simulink model "Three_Stages"  (R2023a)
settings: Solver=FixedStepDiscrete  StartTime=0.0  StopTime=5000  FixedStep=1  RelTol=1e-3
values from neighbouring files (symbols this model uses):
  fw = zeros(16384, 1, 'uint32')    [test.m]
libraries: hdlsllib x27, simulink x27, etargetslib x1
(part 1 of 5)
settings Model: PauseTimes=9  Creator=11983  LastModifiedBy=11983

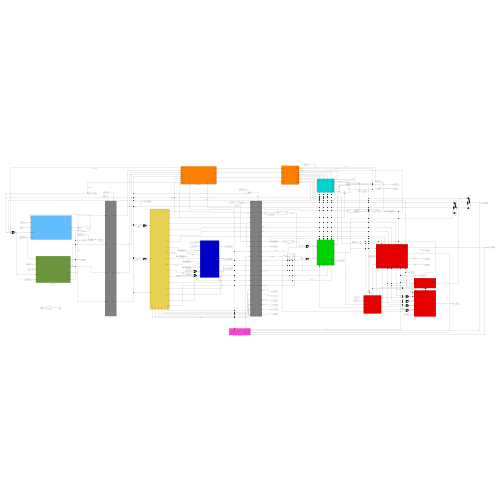
[thumbnail: Simulink's stored preview of the top-level diagram]
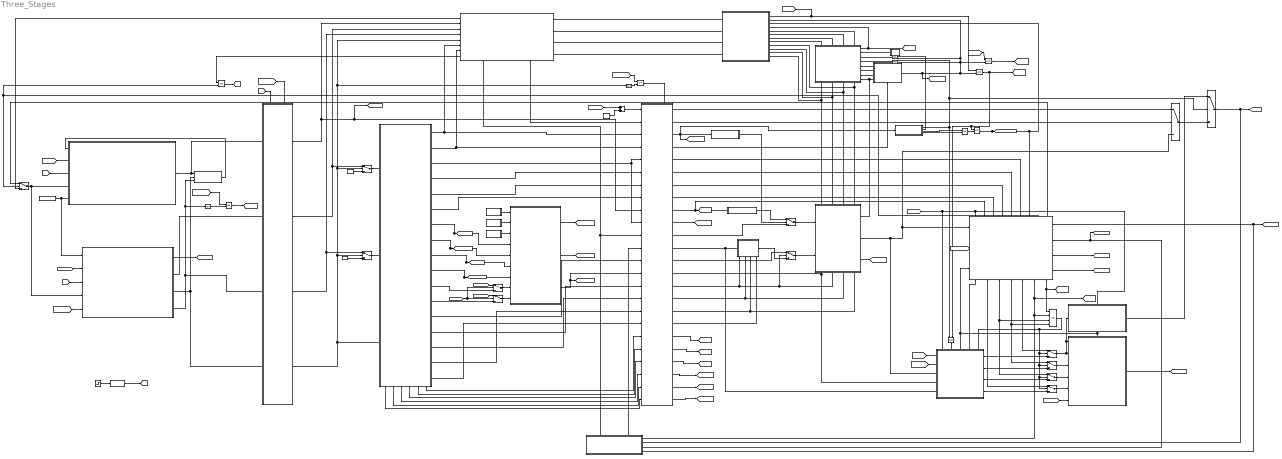
== system Three_Stages ==
  ALU : Subsystem
      settings: PortSchema="{\"entries\":[{\"content\":{\"sides\":[{\"content\":{\"connectorIds\":[\"In1\",\"In2\"]},\"type\":\"ConnectorPlacement.EquallySpacedRectSide\",\"uuid\":\"ccb5df41-1247-48d9-959c-75926096b8fa\"},{\"content\":{\"connectorIds\":[\"In7\",\"Out1\",\"Out2\"],\"side\":\"RIGHT\"},\"type\":\"ConnectorPlacement.EquallySpacedRectSide\",\"uuid\":\"80f2a142-6d0c-48b1-ae68-4f85aa7180f9\"},{\"content\":{\"connectorIds\":[\"Out3\",\"Out4\",\"Out5\",\"Out6\"],\"side\":\"TOP\"},\"type\":\"ConnectorPlacement.EquallySpacedRectSide\",\"uuid\":\"ddd8a3a0-1a29-4746-aba9-d3a66e616423\"},{\"content\":{\"connectorIds\":[\"In3\",\"In4\",\"In5\",\"In6\"],\"side\":\"BOTTOM\"},\"type\":\"ConnectorPlacement.EquallySpacedRectSide\",\"uuid\":\"5581b6e8-dec6-4a13-b9b3-e754e41154dd\"}]},\"type\":\"ConnectorPlacement.EquallySpacedConnector\",\"uuid\":\"f4739204-0172-45d8-8900-7f7503b7c069\"}],\"packageUris\":[\"http://schema.mathworks.com/mf0/Connector/R2020b\"],\"version\":\"1.0\"}"
  APSR : Subsystem
      settings: PortSchema="{\"entries\":[{\"content\":{\"sides\":[{\"content\":{},\"type\":\"ConnectorPlacement.EquallySpacedRectSide\",\"uuid\":\"b04420ff-f19b-4c94-a003-74643939b36f\"},{\"content\":{\"connectorIds\":[\"In5\",\"In6\",\"In7\",\"In8\",\"Out1\",\"Out2\",\"Out3\",\"Out4\"],\"side\":\"RIGHT\"},\"type\":\"ConnectorPlacement.EquallySpacedRectSide\",\"uuid\":\"262487a7-9547-4f2e-9b3b-f72102858df0\"},{\"content\":{\"connectorIds\":[\"Out5\",\"Out6\",\"Out7\",\"Out8\"],\"side\":\"TOP\"},\"type\":\"ConnectorPlacement.EquallySpacedRectSide\",\"uuid\":\"08655cd2-da14-4b4c-a3be-8f888e927bf2\"},{\"content\":{\"connectorIds\":[\"In1\",\"In2\",\"In3\",\"In4\"],\"side\":\"BOTTOM\"},\"type\":\"ConnectorPlacement.EquallySpacedRectSide\",\"uuid\":\"d1ff2338-8405-4e4f-9e8f-6e9f9acda6a4\"}]},\"type\":\"ConnectorPlacement.EquallySpacedConnector\",\"uuid\":\"02373ca2-1c43-4ba4-bf90-ab64c05b49a0\"}],\"packageUris\":[\"http://schema.mathworks.com/mf0/Connector/R2020b\"],\"version\":\"1.0\"}"
  Add : Sum
  Branch_Unit : Subsystem
      settings: PortSchema="{\"entries\":[{\"content\":{\"sides\":[{\"content\":{\"connectorIds\":[\"Out2\",\"In1\",\"In2\",\"In3\",\"In4\",\"In5\",\"In6\",\"Out3\"]},\"type\":\"ConnectorPlacement.EquallySpacedRectSide\",\"uuid\":\"fa39de6f-023a-4353-bbb3-beec0acef9a4\"},{\"content\":{\"connectorIds\":[\"In8\",\"In9\",\"In10\",\"In11\"],\"side\":\"RIGHT\"},\"type\":\"ConnectorPlacement.EquallySpacedRectSide\",\"uuid\":\"2cd56a38-3fbf-451b-a1e9-9297fd516597\"},{\"content\":{\"side\":\"TOP\"},\"type\":\"ConnectorPlacement.EquallySpacedRectSide\",\"uuid\":\"e24db981-f1ca-4813-8aa8-2d70266521c8\"},{\"content\":{\"connectorIds\":[\"In7\",\"Out1\"],\"side\":\"BOTTOM\"},\"type\":\"ConnectorPlacement.EquallySpacedRectSide\",\"uuid\":\"8566e1d9-99e4-42a3-b963-6f1483e5acef\"}]},\"type\":\"ConnectorPlacement.EquallySpacedConnector\",\"uuid\":\"2efaa27e-3a9b-48f9-ab74-8d4ce9e9e835\"}],\"packageUris\":[\"http://schema.mathworks.com/mf0/Connector/R2020b\"],\"version\":\"1.0\"}"
  COND_OK : Subsystem
      settings: PortSchema="{\"entries\":[{\"content\":{\"sides\":[{\"content\":{\"connectorIds\":[\"In1\",\"In2\",\"In3\",\"In4\"]},\"type\":\"ConnectorPlacement.EquallySpacedRectSide\",\"uuid\":\"b7de4efa-7ffd-4508-af86-f3994ca8b638\"},{\"content\":{\"connectorIds\":[\"Out1\"],\"side\":\"RIGHT\"},\"type\":\"ConnectorPlacement.EquallySpacedRectSide\",\"uuid\":\"01c63998-7571-4d66-95c8-a8f2c37a5aa2\"},{\"content\":{\"side\":\"TOP\"},\"type\":\"ConnectorPlacement.EquallySpacedRectSide\",\"uuid\":\"ed1382b1-aa61-428b-a7ef-96829cef3c86\"},{\"content\":{\"connectorIds\":[\"In5\"],\"side\":\"BOTTOM\"},\"type\":\"ConnectorPlacement.EquallySpacedRectSide\",\"uuid\":\"571a99ab-d0c2-4e4e-a524-83c5ee223b5b\"}]},\"type\":\"ConnectorPlacement.EquallySpacedConnector\",\"uuid\":\"3f5959c9-782a-410f-ad4b-6735c3db51ba\"}],\"packageUris\":[\"http://schema.mathworks.com/mf0/Connector/R2020b\"],\"version\":\"1.0\"}"
  Constant : Constant  Value=0  OutDataTypeStr=uint32
  Constant1 : Constant  Value=0
  Constant3 : Constant  Value=0x08000130  VectorParams1D=off
  Constant7 : Constant  Value=4  OutDataTypeStr=uint32
  Data Type Conversion : DataTypeConversion  OutDataTypeStr=boolean  SaturateOnIntegerOverflow=off  RndMeth=Floor
  Forward_Unit : Subsystem
      settings: PortSchema="{\"entries\":[{\"content\":{\"sides\":[{\"content\":{},\"type\":\"ConnectorPlacement.EquallySpacedRectSide\",\"uuid\":\"b518ab8e-5181-4ba3-962c-c49c8d938615\"},{\"content\":{\"connectorIds\":[\"In1\",\"In2\",\"In3\",\"In4\"],\"side\":\"RIGHT\"},\"type\":\"ConnectorPlacement.EquallySpacedRectSide\",\"uuid\":\"5317ce62-8cb4-48f5-b950-79d5c38b61e0\"},{\"content\":{\"connectorIds\":[\"Out1\",\"Out2\"],\"side\":\"TOP\"},\"type\":\"ConnectorPlacement.EquallySpacedRectSide\",\"uuid\":\"43e255fe-bf02-429e-afe6-23a00690485d\"}]},\"type\":\"ConnectorPlacement.EquallySpacedConnector\",\"uuid\":\"73139baf-ff19-4893-8dbb-73622a3eec4b\"}],\"packageUris\":[\"http://schema.mathworks.com/mf0/Connector/R2020b\"],\"version\":\"1.0\"}"
  LDRB_LDRH : Subsystem
      settings: PortSchema="{\"entries\":[{\"content\":{\"sides\":[{\"content\":{\"connectorIds\":[\"In1\"]},\"type\":\"ConnectorPlacement.EquallySpacedRectSide\",\"uuid\":\"1aacb863-4f6f-4fe7-b69a-d5773680006a\"},{\"content\":{\"connectorIds\":[\"Out1\"],\"side\":\"RIGHT\"},\"type\":\"ConnectorPlacement.EquallySpacedRectSide\",\"uuid\":\"1b0cc9e8-d7ed-4611-b678-703fc229f153\"},{\"content\":{\"connectorIds\":[\"In2\"],\"side\":\"TOP\"},\"type\":\"ConnectorPlacement.EquallySpacedRectSide\",\"uuid\":\"6cf80b36-4bc3-4f6e-89b2-b390fea3a693\"},{\"content\":{\"connectorIds\":[\"In3\"],\"side\":\"BOTTOM\"},\"type\":\"ConnectorPlacement.EquallySpacedRectSide\",\"uuid\":\"f50755aa-ce52-486e-b974-6c83f6b16ce4\"}]},\"type\":\"ConnectorPlacement.EquallySpacedConnector\",\"uuid\":\"37988c8b-84fd-4da1-be93-43b2d0148809\"}],\"packageUris\":[\"http://schema.mathworks.com/mf0/Connector/R2020b\"],\"version\":\"1.0\"}"
  LDR_Target : Subsystem
  Logical Operator{1..4,12,14} (6 alike) : Logic  AllPortsSameDT=off  OutDataTypeStr=boolean
  Logical Operator10 : Logic  Operator=OR  Inputs=4  AllPortsSameDT=off  OutDataTypeStr=boolean
  Logical Operator15 : Logic  Operator=NOT  AllPortsSameDT=off  OutDataTypeStr=boolean
  Logical Operator{5..6,21..22} (4 alike) : Logic  Operator=OR  AllPortsSameDT=off  OutDataTypeStr=boolean
  Logical Operator23 : Logic  Operator=NOT  AllPortsSameDT=off  OutDataTypeStr=boolean
  MR : Subsystem
      settings: PortSchema="{\"entries\":[{\"content\":{\"sides\":[{\"content\":{\"connectorIds\":[\"In1\",\"In2\",\"In3\"]},\"type\":\"ConnectorPlacement.EquallySpacedRectSide\",\"uuid\":\"ae034d06-3b44-4ece-97be-40f77d25c887\"},{\"content\":{\"connectorIds\":[\"Out1\",\"Out2\",\"Out3\",\"Out4\"],\"side\":\"RIGHT\"},\"type\":\"ConnectorPlacement.EquallySpacedRectSide\",\"uuid\":\"97e4f072-c582-4d8b-a0d0-105be19de914\"},{\"content\":{\"connectorIds\":[\"In4\",\"In5\",\"In6\",\"In7\",\"In8\",\"In9\",\"In10\",\"Out12\",\"Out13\"],\"side\":\"TOP\"},\"type\":\"ConnectorPlacement.EquallySpacedRectSide\",\"uuid\":\"0c52d681-aa90-4260-97f0-099fed25df92\"},{\"content\":{\"connectorIds\":[\"Out5\",\"Out6\",\"Out7\",\"Out8\",\"Out9\",\"Out10\",\"Out11\"],\"side\":\"BOTTOM\"},\"type\":\"ConnectorPlacement.EquallySpacedRectSide\",\"uuid\":\"f0439111-5f7c-4712-89ea-153c665c0054\"}]},\"type\":\"ConnectorPlacement.EquallySpacedConnector\",\"uuid\":\"3d8c92c8-6a6f-4c3f-a3c8-33ac8d15b626\"}],\"packageUris\":[\"http://schema.mathworks.com/mf0/Connector/R2020b\"],\"version\":\"1.0\"}"
  PC : Subsystem
  Prefetch_Unit : Subsystem
  Register File : Subsystem
  STRB_STRH : Subsystem
      settings: PortSchema="{\"entries\":[{\"content\":{\"sides\":[{\"content\":{\"connectorIds\":[\"In1\",\"In2\",\"In3\",\"In4\",\"In5\"]},\"type\":\"ConnectorPlacement.EquallySpacedRectSide\",\"uuid\":\"52cc573e-20cd-47d9-80c8-fb5377adebe3\"},{\"content\":{\"connectorIds\":[\"Out1\",\"Out2\",\"Out3\",\"Out4\"],\"side\":\"RIGHT\"},\"type\":\"ConnectorPlacement.EquallySpacedRectSide\",\"uuid\":\"a4a5e072-7857-4af3-85db-797d3693bf36\"},{\"content\":{\"connectorIds\":[\"In6\",\"In7\",\"In8\",\"In9\",\"In10\"],\"side\":\"TOP\"},\"type\":\"ConnectorPlacement.EquallySpacedRectSide\",\"uuid\":\"ea3ffc43-3311-4906-a9ee-9debdf9ad28c\"},{\"content\":{\"side\":\"BOTTOM\"},\"type\":\"ConnectorPlacement.EquallySpacedRectSide\",\"uuid\":\"e3f27f00-6d88-4589-b3c9-a064ef027647\"}]},\"type\":\"ConnectorPlacement.EquallySpacedConnector\",\"uuid\":\"664d1095-24c2-4b6b-a161-99b2f71d747b\"}],\"packageUris\":[\"http://schema.mathworks.com/mf0/Connector/R2020b\"],\"version\":\"1.0\"}"
  Step : Step  Time=2.2  SampleTime=1
  Subsystem1 : Subsystem
      settings: PortSchema="{\"entries\":[{\"content\":{\"sides\":[{\"content\":{\"connectorIds\":[\"In1\",\"In2\",\"In3\",\"In4\"]},\"type\":\"ConnectorPlacement.EquallySpacedRectSide\",\"uuid\":\"b636389a-7517-44e7-b701-adf22a5dae08\"},{\"content\":{\"connectorIds\":[\"Out1\",\"Out2\",\"Out3\",\"Out4\"],\"side\":\"RIGHT\"},\"type\":\"ConnectorPlacement.EquallySpacedRectSide\",\"uuid\":\"a093e9de-de32-4ec9-9bcc-d63488a9f5df\"},{\"content\":{\"connectorIds\":[\"In5\",\"In6\"],\"side\":\"TOP\"},\"type\":\"ConnectorPlacement.EquallySpacedRectSide\",\"uuid\":\"0686ded3-feaa-49de-a1b1-14e15ce2ab70\"}]},\"type\":\"ConnectorPlacement.EquallySpacedConnector\",\"uuid\":\"33f9a1b7-843e-4ab1-9626-193f0cb3215d\"}],\"packageUris\":[\"http://schema.mathworks.com/mf0/Connector/R2020b\"],\"version\":\"1.0\"}"
  Subsystem13 : Subsystem
      settings: PortSchema="{\"entries\":[{\"content\":{\"sides\":[{\"content\":{\"connectorIds\":[\"In1\"]},\"type\":\"ConnectorPlacement.EquallySpacedRectSide\",\"uuid\":\"4653521f-c5b0-44ee-87bd-1e9a678c2349\"},{\"content\":{\"connectorIds\":[\"Out1\"],\"side\":\"RIGHT\"},\"type\":\"ConnectorPlacement.EquallySpacedRectSide\",\"uuid\":\"2d3a92f1-c2bf-4739-8a2e-22a17e3c5465\"},{\"content\":{\"side\":\"TOP\"},\"type\":\"ConnectorPlacement.EquallySpacedRectSide\",\"uuid\":\"dec91679-c767-4ffa-aded-7a717f01530d\"},{\"content\":{\"connectorIds\":[\"In2\",\"In3\",\"In4\",\"In5\"],\"side\":\"BOTTOM\"},\"type\":\"ConnectorPlacement.EquallySpacedRectSide\",\"uuid\":\"b2049017-66dd-4d9f-8220-bbbb14711246\"}]},\"type\":\"ConnectorPlacement.EquallySpacedConnector\",\"uuid\":\"86f521a6-6afa-4d7d-9bc3-b40505ae83a4\"}],\"packageUris\":[\"http://schema.mathworks.com/mf0/Connector/R2020b\"],\"version\":\"1.0\"}"
  Subsystem2 : Subsystem
      settings: PortSchema="{\"entries\":[{\"content\":{\"sides\":[{\"content\":{\"connectorIds\":[\"In1\",\"In2\",\"In3\"]},\"type\":\"ConnectorPlacement.EquallySpacedRectSide\",\"uuid\":\"37376870-fc31-46e0-82d0-6de34bc1bd49\"},{\"content\":{\"connectorIds\":[\"Out1\",\"Out2\",\"Out3\",\"Out4\",\"Out5\",\"Out6\",\"Out7\",\"Out8\",\"Out9\",\"Out10\",\"Out11\",\"Out12\",\"Out13\",\"Out14\",\"Out15\",\"Out16\",\"Out17\"],\"side\":\"RIGHT\"},\"type\":\"ConnectorPlacement.EquallySpacedRectSide\",\"uuid\":\"240ad313-7487-41b8-b4f3-25aa4e288c60\"},{\"content\":{\"side\":\"TOP\"},\"type\":\"ConnectorPlacement.EquallySpacedRectSide\",\"uuid\":\"4c57ba5a-1bd7-4c75-853e-e9f9b7d7373d\"},{\"content\":{\"connectorIds\":[\"Out18\",\"Out19\",\"Out20\",\"Out21\",\"Out22\",\"Out23\"],\"side\":\"BOTTOM\"},\"type\":\"ConnectorPlacement.EquallySpacedRectSide\",\"uuid\":\"b2a89158-f928-4e03-8a4f-4307562c8f8b\"}]},\"type\":\"ConnectorPlacement.EquallySpacedConnector\",\"uuid\":\"be61e4cd-4b1f-4051-8408-66a432478836\"}],\"packageUris\":[\"http://schema.mathworks.com/mf0/Connector/R2020b\"],\"version\":\"1.0\"}"
  Subsystem21 : Subsystem
      settings: PortSchema="{\"entries\":[{\"content\":{\"sides\":[{\"content\":{\"connectorIds\":[\"In1\",\"In2\",\"In3\",\"In4\",\"In5\",\"In6\",\"In7\",\"In8\",\"In9\",\"In10\",\"In11\",\"In12\",\"In13\",\"In14\",\"In15\",\"In16\",\"In17\",\"In18\",\"In19\",\"In20\",\"In21\",\"In22\",\"In23\",\"In24\"]},\"type\":\"ConnectorPlacement.EquallySpacedRectSide\",\"uuid\":\"4b7059a5-6288-49ad-9997-b62eea665d5e\"},{\"content\":{\"connectorIds\":[\"Out1\",\"Out2\",\"Out3\",\"Out4\",\"Out5\",\"Out6\",\"Out7\",\"Out8\",\"Out9\",\"Out10\",\"Out11\",\"Out12\",\"Out13\",\"Out14\",\"Out15\",\"Out16\",\"Out17\",\"Out18\",\"Out19\",\"Out20\",\"Out21\",\"Out22\",\"Out23\",\"Out24\"],\"side\":\"RIGHT\"},\"type\":\"ConnectorPlacement.EquallySpacedRectSide\",\"uuid\":\"a56c66a4-1870-4e19-94f9-e8042e703f05\"},{\"content\":{\"connectorIds\":[\"In25\",\"In26\"],\"side\":\"TOP\"},\"type\":\"ConnectorPlacement.EquallySpacedRectSide\",\"uuid\":\"7f424b6d-78e9-4b64-bd47-1686fcb53e5c\"},{\"content\":{\"side\":\"BOTTOM\"},\"type\":\"ConnectorPlacement.EquallySpacedRectSide\",\"uuid\":\"2e30f2a8-cee4-43cc-adcf-6850d631dff2\"}]},\"type\":\"ConnectorPlacement.EquallySpacedConnector\",\"uuid\":\"bb030113-0317-44c2-9b6f-777570308f9b\"}],\"packageUris\":[\"http://schema.mathworks.com/mf0/Connector/R2020b\"],\"version\":\"1.0\"}"
  Subsystem3 : Subsystem
  Subsystem4 : Subsystem
  Subsystem5 : Subsystem
  Subsystem7 : Subsystem
  Subsystem8 : Subsystem
  Subsystem9 : Subsystem
  Switch{,1..4,10..11,13} (8 alike) : Switch  Criteria=u2 ~= 0  SaturateOnIntegerOverflow=off  InputSameDT=off
  Switch12 : Switch  Criteria=u2 > Threshold  SaturateOnIntegerOverflow=off  InputSameDT=off
  Switch5 : Switch  Criteria=u2 ~= 0  OutDataTypeStr=uint32  SaturateOnIntegerOverflow=off  InputSameDT=off
  Switch6 : Switch  Criteria=u2 ~= 0  OutDataTypeStr=boolean  SaturateOnIntegerOverflow=off  InputSameDT=off
  Switch7 : Switch  Criteria=u2 ~= 0  OutDataTypeStr=boolean  SaturateOnIntegerOverflow=off  InputSameDT=off
  Switch8 : Switch  Criteria=u2 ~= 0  OutDataTypeStr=uint32  SaturateOnIntegerOverflow=off  InputSameDT=off
  i : Subsystem
  id_pc_val2 : Subsystem
  memory : Subsystem
      settings: PortSchema="{\"entries\":[{\"content\":{\"sides\":[{\"content\":{\"connectorIds\":[\"In1\",\"In2\",\"In3\",\"In4\",\"In5\",\"In6\"]},\"type\":\"ConnectorPlacement.EquallySpacedRectSide\",\"uuid\":\"1e789dec-d403-461e-8d45-ab9493bc7df3\"},{\"content\":{\"connectorIds\":[\"Out1\"],\"side\":\"RIGHT\"},\"type\":\"ConnectorPlacement.EquallySpacedRectSide\",\"uuid\":\"863b6fcc-e8ea-4978-9b45-60c5471a4665\"},{\"content\":{\"connectorIds\":[\"Out2\"],\"side\":\"TOP\"},\"type\":\"ConnectorPlacement.EquallySpacedRectSide\",\"uuid\":\"b83e2490-8135-444c-8ad0-08dab006a2c6\"}]},\"type\":\"ConnectorPlacement.EquallySpacedConnector\",\"uuid\":\"749f8af8-7b61-4e19-bb32-412ba8347444\"}],\"packageUris\":[\"http://schema.mathworks.com/mf0/Connector/R2020b\"],\"version\":\"1.0\"}"
  tag scope: alu_result_hi=global, ex_WB_addr=global, ex_WB_en=global, ex_WB_en_eff=global, ex_cond_ok=global, ex_instr_addr=global, ex_is_multi_op=global, ex_opcode=global, ex_rd_hi=global, ex_rd_lo=global, ex_s=global, ex_two_wb=global, ex_valid=global, ex_valid_eff=global, flush=global, ic_data=global, id_read_addr_1=global, id_read_addr_2=global, id_read_data_1=global, id_read_data_2=global, id_read_en_1=global, id_read_en_2=global, if_id_addr=global, if_id_stall=global, mr_busy=global, mr_rf_addr=global, mr_rf_rd_addr=global, mr_rf_rd_data=global, mr_rf_rd_en=global, mr_rf_wdata=global, mr_rf_we=global, pf_fetch_pc=global, rf_wdata=global, rst_n=global
  wires:
  Subsystem21/11(data_1_out) -> Switch10/3  "ex_data_1"
  Switch4/1 -> ALU/2(alu_b)  "alu_b"
  APSR/4(apsr_c) -> ALU/7(alu_carry_in), COND_OK/4(cf)  "apsr_c"
  Subsystem21/16(alu_shamt_out) -> Subsystem13/3(alu_shamt_out), ALU/5(alu_shamt)  "ex_alu_shamt"
  [flush] -> Subsystem1/5(In4)
  Subsystem1/2(instr) -> Branch_Unit/2(id_instr), Switch/1  "if_id_instr"
  Constant/1 -> Switch/3
  Constant1/1 -> Switch1/3
  Subsystem1/3(id_instr1) -> Switch1/1, Branch_Unit/3(id_instr1)  "instr_width_out"
  Switch/1 -> Subsystem2/1(instr)
  Switch1/1 -> Subsystem2/2(instr_width)
  Subsystem2/1(opcode) -> Subsystem21/3(opcode_in), Branch_Unit/5(id_instr5)  "id_opcode"
  Subsystem2/4(rn) -> Subsystem21/6(rn_in)
  Subsystem2/5(rm) -> Subsystem21/7(rm_in)
  Subsystem2/13(imm32) -> Subsystem21/13(imm32_in)  "id_imm32"
  Subsystem2/8(read_addr_1) -> Register File/5(read_addr_1), [id_read_addr_1]  "id_read_addr_1"
  Subsystem2/7(read_en_1) -> Register File/4(read_en_1), [id_read_en_1]  "read_en_1"
  Subsystem2/10(read_addr_2) -> Register File/7(read_addr_2), [id_read_addr_2]  "id_read_addr_2"
  Subsystem2/9(read_en_2) -> Register File/6(read_en_2), [id_read_en_2]  "id_read_en_2"
  Subsystem2/23(write_en) -> Subsystem21/19(WB_en_in)
  Subsystem2/16(alu_op) -> Subsystem21/17(alu_op_in)
  Subsystem2/14(alu_src_b) -> Subsystem21/15(alu_src_b_in)
  Subsystem2/15(alu_shamt) -> Subsystem21/16(alu_shamt_in)
  Subsystem2/17(alu_shift_type) -> Subsystem21/18(alu_shift_type_in)
  Subsystem2/6(reg_list) -> Subsystem21/8(reg_list_in)  "id_reg_list"
  Subsystem21/15(alu_src_b_out) -> Subsystem13/2(alu_src_b_out), Switch4/2, ALU/4(alu_src_b)  "alu_src_b_out"
  Subsystem21/13(imm32_out) -> Switch4/1  "ex_imm32"
  Subsystem21/17(alu_op_out) -> Subsystem13/4(alu_shamt_out1), ALU/6(alu_op)  "alu_op_out"
  Subsystem21/4(cond_out) -> COND_OK/5(cond_out)  "ex_cond"
  [ex_WB_en] -> Logical Operator4/1  "ex_WB_en"
  COND_OK/1(Out1) -> [ex_cond_ok], Logical Operator4/2, Subsystem5/2(In5), Logical Operator14/2, Logical Operator12/2, Logical Operator3/2  "ex_cond_ok"
  Logical Operator4/1 -> [ex_WB_en_eff]  "ex_WB_en_eff"
  ALU/6(alu_n) -> APSR/4(alu_n), Subsystem5/9(alu_n)  "alu_n"
  ALU/5(alu_z) -> Subsystem5/10(alu_z), APSR/3(alu_z)  "alu_z"
  ALU/4(alu_v) -> Subsystem5/11(alu_v), APSR/2(alu_v)  "alu_v"
  ALU/3(alu_c) -> Subsystem5/12(alu_c), APSR/1(alu_c)  "alu_c"
  APSR/1(apsr_v) -> COND_OK/1(apsr_v)
  APSR/2(apsr_z) -> COND_OK/2(z)
  APSR/3(apsr_n) -> COND_OK/3(apsr_n)
  Subsystem21/3(opcode_out) -> i/1(opcode), [ex_opcode], Subsystem3/1(ex_opcode)  "ex_opcode"
  Subsystem21/21(valid_out) -> [ex_valid]  "ex_valid"
  [ex_valid] -> Logical Operator3/1, Subsystem5/1(In2)  "ex_valid"
  Subsystem21/19(WB_en) -> [ex_WB_en]  "ex_WB_en"
  Logical Operator2/1 -> STRB_STRH/7(In6)  "ex_mem_rd_eff"
  Logical Operator3/1 -> [ex_valid_eff], Logical Operator1/1, Logical Operator2/2  "ex_valid_eff"
  Logical Operator6/1 -> Logical Operator1/2
  Logical Operator1/1 -> Subsystem5/3(In6), MR/10(In1), [ex_is_multi_op]  "ex_is_multi_op_raw"
  MR/11(busy) -> [mr_busy], Logical Operator10/1  "mr_busy"
  Switch5/1 -> memory/1(read_addr), LDRB_LDRH/1(In1), memory/2(write_addr)  "mem_addr_int"
  [pf_fetch_pc] -> memory/6(instr_addr)  "pf_fetch_pc"
  memory/2(read_data) -> MR/3(rst_n9), STRB_STRH/8(mem_rdata), LDRB_LDRH/3(read_data)  "mem_rdata_int"
  memory/1(instr_data) -> [ic_data]  "ic_data"
  Logical Operator10/1 -> Switch6/2, Switch7/2, Switch8/2, Switch5/2, STRB_STRH/10(In1)  "mr_port_active"
  Subsystem21/10(WB_addr_out) -> [ex_WB_addr]  "ex_WB_addr"
  MR/9(mem_addr) -> Switch5/1  "mr_mem_addr"
  MR/8(mem_re) -> Logical Operator10/4, Switch6/1  "mr_mem_re"
  MR/7(mem_we) -> Logical Operator10/3, Switch7/1  "mr_mem_we"
  MR/6(mem_wdata) -> Switch8/1  "mr_mem_wdata"
  Subsystem21/12(data_2_out) -> STRB_STRH/5(ex_data_2), Subsystem13/1(data_2_out)  "ex_data_2"
  Switch6/1 -> memory/3(read_en)  "mem_re_int"
  Switch7/1 -> memory/4(write_en)  "mem_we_int"
  Switch8/1 -> memory/5(write_data)  "mem_wdata_int"
  Subsystem21/8(reg_list_out) -> MR/6(rst_n5)  "ex_reg_list"
  Subsystem4/1(Out1) -> APSR/6(valid)  "apsr_valid"
  Subsystem21/20(s_out) -> [ex_s]  "ex_s"
  [ex_s] -> Subsystem5/4(In4), APSR/5(s)  "ex_s"
  Subsystem3/1(ex_is_load) -> Logical Operator12/1, Switch13/2, Logical Operator2/1  "ex_is_load"
  Subsystem3/2(ex_is_store) -> Logical Operator14/1  "ex_is_store"
  Subsystem3/3(ex_is_multi_ld) -> Logical Operator6/1
  Subsystem3/4(ex_is_multi_st) -> Logical Operator6/2
  Logical Operator12/1 -> APSR/8(is_load)
  Logical Operator14/1 -> APSR/7(is_store)
  Subsystem2/3(rd) -> Subsystem21/5(rd_in), Subsystem21/10(WB_addr_in)
  MR/10(rf_we) -> [mr_rf_we], Logical Operator10/2, Forward_Unit/1(mr_rf_we)  "mr_rf_we"
  MR/1(rf_addr) -> [mr_rf_addr], Forward_Unit/4(mr_rf_addr)  "mr_rf_addr"
  MR/2(rf_wdata) -> [mr_rf_wdata], Forward_Unit/3(mr_rf_wdata)  "mr_rf_wdata"
  MR/3(rf_rd_addr) -> [mr_rf_rd_addr]  "mr_rf_rd_addr"
  [mr_rf_rd_addr] -> Switch12/1
  [mr_rf_rd_en] -> Switch11/1  "mr_rf_rd_en"
  MR/4(rf_rd_en) -> [mr_rf_rd_en]  "mr_rf_rd_en"
  [ic_data] -> Prefetch_Unit/2(instr_data)
  [flush] -> Prefetch_Unit/3(instr_data2)  "flush"
  Switch2/1 -> Prefetch_Unit/4(instr_data3), PC/4(In5)  "flush_target"
  [pipeline_stall] -> Prefetch_Unit/5(instr_data4)
  Prefetch_Unit/1(Out1) -> [pf_fetch_pc]  "pf_fetch_pc"
  Prefetch_Unit/2(Out2) -> Subsystem1/2(In1)  "pf_instr"
  Prefetch_Unit/3(Out3) -> id_pc_val2/2(In4), Subsystem1/4(In16)  "pf_width"
  Prefetch_Unit/4(Out4) -> Logical Operator15/1, id_pc_val2/3(In5), Subsystem1/3(In2)  "pf_pop_valid"
  Constant3/1 -> PC/5(In6), Prefetch_Unit/1(In2)
  i/1(Out3) -> Switch10/2  "ex_need_pc"
  [if_id_stall] -> PC/2(In2)
  PC/1(Out1) -> Subsystem1/1(In6), id_pc_val2/1(In1)  "pc_addr"
  [flush] -> PC/3(In4)
  id_pc_val2/1(Out1) -> PC/1(In1)
  Subsystem1/1(id_instr3) -> [if_id_addr], Subsystem21/9(instr_addr_in), Branch_Unit/1(id_instr3)  "id_instr_addr"
  Logical Operator21/1 -> [flush]  "flush"
  Branch_Unit/3(Out1) -> Logical Operator21/1  "branch_taken"
  MR/12(load_pc_en) -> Logical Operator21/2, Switch2/2  "mr_load_pc_en"
  MR/13(load_pc_val) -> Switch2/1  "mr_load_pc_val"
  Branch_Unit/2(Out2) -> Switch2/3  "branch_target"
  Branch_Unit/1(link_en_in) -> Subsystem21/2(link_en_in)
  Subsystem21/2(link_en_out) -> Switch3/2  "link_en_out"
  Switch3/1 -> Switch13/3
  Subsystem21/1(link_pc_out) -> Switch3/1  "link_pc_out"
  LDRB_LDRH/1(Out1) -> Switch13/1
  Switch13/1 -> [rf_wdata], Forward_Unit/2(rf_wdata)  "rf_wdata"
  Subsystem1/4(instr_valid) -> Branch_Unit/4(id_instr4), Logical Operator23/1, Switch/2, Switch1/2, Subsystem2/3(if_id_valid)  "if_id_valid"
  Logical Operator23/1 -> Logical Operator22/2
  [pipeline_stall] -> Logical Operator22/1
  Logical Operator22/1 -> Subsystem21/26(stall)  "id_ex_stall"
  Subsystem2/2(cond) -> Branch_Unit/6(id_instr6), Subsystem21/4(cond_in)  "id_cond"
  Subsystem5/1(id_instr8) -> Branch_Unit/8(id_instr8)
  Subsystem5/2(id_instr9) -> Branch_Unit/9(id_instr9)
  Subsystem5/3(id_instr10) -> Branch_Unit/10(id_instr10)
  Subsystem5/4(id_instr11) -> Branch_Unit/11(id_instr11)
  APSR/8(fwd_n) -> Subsystem5/5(fwd_n)
  APSR/7(fwd_z) -> Subsystem5/6(fwd_z)
  APSR/6(fwd_v) -> Subsystem5/7(fwd_v)
  APSR/5(fwd_c) -> Subsystem5/8(fwd_c)  "fwd_c"
  Subsystem21/5(rd_out) -> MR/9(rst_n6)  "ex_rd"
  Subsystem21/7(rm_out) -> MR/7(rst_n7)  "rm_out"
  ALU/1(alu_result) -> STRB_STRH/3(alu_result), Switch3/3, MR/1(rst_n3)  "base"
  Subsystem21/6(rn_out) -> MR/8(rst_n4)  "base_reg"
  Register File/3(alu_acc_in) -> [mr_rf_rd_data], Subsystem21/14(alu_acc_in)  "mr_rf_rd_data"
  Register File/1(Out1) -> [id_read_data_1]  "id_read_data_1"
  Register File/2(Out2) -> [id_read_data_2]  "id_read_data_2"
  Subsystem2/22(s) -> Subsystem21/20(s_in)
  Subsystem2/21(valid) -> Subsystem21/21(valid_in)
  [mr_rf_rd_data] -> MR/2(rst_n10)
  Step/1 -> Data Type Conversion/1  "rst_n"
  Data Type Conversion/1 -> [rst_n]
  Add/1 -> Subsystem21/1(link_pc_in)
  [if_id_addr] -> Add/1  "if_id_addr"
  Constant7/1 -> Add/2
  Subsystem7/1(rf_we_int) -> Register File/3(rf_we_int)  "rf_we_int"
  Subsystem8/1(rf_we_addr_int) -> Register File/2(In3)  "rf_we_addr_int"
  Subsystem9/1(rf_wdata_int) -> Register File/1(In2)  "rf_wdata_int"
  Subsystem21/9(instr_addr_out) -> MR/5(instr_addr_out), LDR_Target/1(ex_instr_addr), [ex_instr_addr]  "ex_instr_addr"
  Switch10/1 -> ALU/1(alu_a)  "alu_a"
  [mr_busy] -> Switch11/2, Switch12/2  "mr_busy"
  Subsystem2/11(ra_valid) -> Switch11/3  "id_ra_valid"
  Subsystem2/12(ra) -> Switch12/3  "id_ra"
  Switch11/1 -> Register File/8(In11)  "read_en_3"
  Switch12/1 -> Register File/9(In13)  "read_addr_3"
  Subsystem21/14(alu_acc_out) -> STRB_STRH/4(mem_rdata1), ALU/3(alu_acc)
  Subsystem2/20(rd_lo) -> Subsystem21/22(rd_lo_in)
  Subsystem2/19(rd_hi) -> Subsystem21/23(rd_hi_in)
  Subsystem2/18(two_wb) -> Subsystem21/24(two_wb_in)  "id_two_wb"
  Subsystem21/22(rd_lo_out) -> [ex_rd_lo]  "ex_rd_lo"
  Subsystem21/23(rd_hi_out) -> [ex_rd_hi]  "ex_rd_hi"
  Subsystem21/24(two_wb_out) -> [ex_two_wb]  "ex_two_wb"
  ALU/2(alu_result_hi) -> [alu_result_hi]
  Logical Operator5/1 -> [if_id_stall]  "if_id_stall"
  [pipeline_stall] -> Logical Operator5/1
  Logical Operator15/1 -> Logical Operator5/2  "if_id_stall"
  [pipeline_stall] -> Subsystem1/6(In3)  "if_id_stall"
  [ex_opcode] -> LDRB_LDRH/2(In3), MR/4(rst_n1), STRB_STRH/6(In3)
  [ex_valid] -> STRB_STRH/1(In4)  "ex_valid"
  [ex_cond_ok] -> STRB_STRH/2(In5)
  STRB_STRH/1(Out4) -> Switch5/3
  STRB_STRH/2(Out2) -> Switch6/3
  STRB_STRH/3(Out3) -> Switch7/3
  STRB_STRH/4(Out5) -> Switch8/3
  Subsystem13/1(Out1) -> Switch4/3
  Subsystem21/18(alu_shift_type_out) -> Subsystem13/5(alu_shamt_out2)  "alu_shift_type_out"
  MR/5(mr_start) -> STRB_STRH/9(mr_start)
  LDR_Target/1(ldr_target) -> Switch10/1
  Forward_Unit/1(id_ex_data_1_in) -> Branch_Unit/7(id_instr7), Subsystem21/11(data_1_in)
  Forward_Unit/2(id_ex_data_2_in) -> Subsystem21/12(data_2_in)

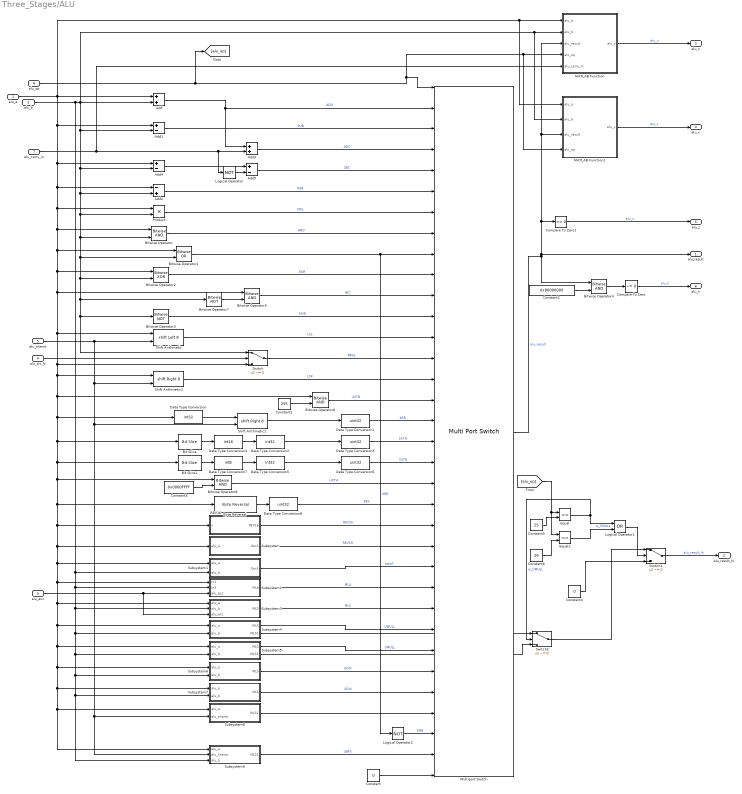
== system Three_Stages/ALU ==
  alu_a : Inport
  alu_b : Inport  Port=2
  alu_acc : Inport  Port=3
  alu_src_b : Inport  Port=4
  alu_shamt : Inport  Port=5
  alu_op : Inport  Port=6
  alu_carry_in : Inport  Port=7
  Add : Sum  OutDataTypeStr=uint32
  Add1 : Sum  Inputs=+-  OutDataTypeStr=uint32
  Add2 : Sum  Inputs=-+  OutDataTypeStr=uint32
  Add3 : Sum  OutDataTypeStr=uint32
  Add4 : Sum  Inputs=+-  OutDataTypeStr=uint32
  Add5 : Sum  Inputs=+-  OutDataTypeStr=uint32
  Bit Slice : hdlsllib/Logic and Bit Operations/Bit Slice  lidx=15  ridx=0
  Bit Slice1 : hdlsllib/Logic and Bit Operations/Bit Slice  lidx=7  ridx=0
  Bitwise Operator{,4..6} (4 alike) : simulink/Logic and Bit Operations/Bitwise Operator  logicop=AND  UseBitMask=off  NumInputPorts=2  BitMask=bin2dec('11011001')  BitMaskRealWorld=Stored Integer
  Bitwise Operator1 : simulink/Logic and Bit Operations/Bitwise Operator  logicop=OR  UseBitMask=off  NumInputPorts=2  BitMask=bin2dec('11011001')  BitMaskRealWorld=Stored Integer
  Bitwise Operator2 : simulink/Logic and Bit Operations/Bitwise Operator  logicop=XOR  UseBitMask=off  NumInputPorts=2  BitMask=bin2dec('11011001')  BitMaskRealWorld=Stored Integer
  Bitwise Operator3 : simulink/Logic and Bit Operations/Bitwise Operator  logicop=NOT  UseBitMask=off  BitMask=bin2dec('11011001')  BitMaskRealWorld=Stored Integer
  Bitwise Operator7 : simulink/Logic and Bit Operations/Bitwise Operator  logicop=NOT  UseBitMask=off  BitMask=bin2dec('11011001')  BitMaskRealWorld=Stored Integer
  Bitwise Operator8 : simulink/Logic and Bit Operations/Bitwise Operator  logicop=AND  UseBitMask=off  NumInputPorts=2  BitMask=0x0000FFFF  BitMaskRealWorld=Stored Integer
  Byte Reversal : etargetslib/Byte Reversal  numInp=1
      settings: LibrarySourceBlock=embeddedtargetslib/Host Communication/Byte Reversal
  Compare To Zero : simulink/Logic and Bit Operations/Compare To Zero  relop=~=  OutDataTypeStr=boolean
  Compare To Zero1 : simulink/Logic and Bit Operations/Compare To Zero  relop===  OutDataTypeStr=boolean
  Constant : Constant  Value=0  OutDataTypeStr=uint32
  Constant1 : Constant  Value=255  OutDataTypeStr=uint32
  Constant2 : Constant  Value=0x80000000  OutDataTypeStr=uint32
  Constant3 : Constant  Value=0x0000FFFF
  Constant4 : Constant  Value=0
  Constant5 : Constant  Value=25
  Constant6 : Constant  Value=26
  Data Type Conversion : DataTypeConversion  OutDataTypeStr=int32  SaturateOnIntegerOverflow=off  RndMeth=Floor
  Data Type Conversion{1,3,6,8} (4 alike) : DataTypeConversion  OutDataTypeStr=uint32  SaturateOnIntegerOverflow=off  RndMeth=Floor
  Data Type Conversion2 : DataTypeConversion  OutDataTypeStr=int32  SaturateOnIntegerOverflow=off  RndMeth=Floor
  Data Type Conversion4 : DataTypeConversion  OutDataTypeStr=int16  SaturateOnIntegerOverflow=off  RndMeth=Floor
  Data Type Conversion5 : DataTypeConversion  OutDataTypeStr=int32  SaturateOnIntegerOverflow=off  RndMeth=Floor
  Data Type Conversion7 : DataTypeConversion  OutDataTypeStr=int8  SaturateOnIntegerOverflow=off  RndMeth=Floor
  Equal : RelationalOperator  Operator===  OutDataTypeStr=boolean  RndMeth=Simplest  InputSameDT=off
  Equal1 : RelationalOperator  Operator===  OutDataTypeStr=boolean  RndMeth=Simplest  InputSameDT=off
  Logical Operator : Logic  Operator=NOT  AllPortsSameDT=off  OutDataTypeStr=boolean
  Logical Operator1 : Logic  Operator=OR  AllPortsSameDT=off  OutDataTypeStr=boolean
  Logical Operator2 : Logic  Operator=NOT  AllPortsSameDT=off  OutDataTypeStr=boolean
  MATLAB Function : MATLAB Function  TreatAsAtomicUnit=on
  MATLAB Function1 : MATLAB Function  TreatAsAtomicUnit=on
  Multiport Switch : MultiPortSwitch  DataPortOrder=Zero-based contiguous  Inputs=32  DataPortForDefault=Additional data port  zeroidx=on  OutDataTypeStr=uint32  SaturateOnIntegerOverflow=off  InputSameDT=off
  Product : Product  OutDataTypeStr=uint32
  REV16 : Subsystem
  Shift Arithmetic : ArithShift  BitShiftNumberSource=Input port  BitShiftNumber=8  BitShiftDirection=Left
      settings: InputPortMap=u0,p1
  Shift Arithmetic1 : ArithShift  BitShiftNumberSource=Input port  BitShiftNumber=8  BitShiftDirection=Right
      settings: InputPortMap=u0,p1
  Shift Arithmetic2 : ArithShift  BitShiftNumberSource=Input port  BitShiftNumber=8  BitShiftDirection=Right
      settings: InputPortMap=u0,p1
  Subsystem : Subsystem
  Subsystem1 : Subsystem
  Subsystem2 : Subsystem
  Subsystem3 : Subsystem
  Subsystem4 : Subsystem
  Subsystem5 : Subsystem
  Subsystem6 : Subsystem
  Subsystem7 : Subsystem
  Subsystem8 : Subsystem
  Subsystem9 : Subsystem
  Switch : Switch  Criteria=u2 ~= 0  OutDataTypeStr=uint32  SaturateOnIntegerOverflow=off  InputSameDT=off
  Switch1 : Switch  Criteria=u2 ~= 0  SaturateOnIntegerOverflow=off  InputSameDT=off
  Switch2 : Switch  Criteria=u2 ~= 0  SaturateOnIntegerOverflow=off  InputSameDT=off
  alu_result : Outport
  alu_result_hi : Outport  Port=2
  alu_c : Outport  Port=3  OutDataTypeStr=boolean
  alu_v : Outport  Port=4  OutDataTypeStr=boolean
  alu_z : Outport  Port=5
  alu_n : Outport  Port=6
  wires:
  alu_op/1 -> [alu_op], MATLAB Function1/4(alu_op), MATLAB Function/4(alu_op), Multiport Switch/1
  alu_b/1 -> Subsystem9/3(alu_b), Subsystem7/2(alu_b), Subsystem6/2(alu_b), Subsystem5/2(alu_b), Subsystem4/2(alu_b), Subsystem3/2(alu_b), Subsystem2/2(In2), Subsystem1/2(alu_b), MATLAB Function1/2(alu_b), MATLAB Function/2(alu_b), Bitwise Operator7/1, Bitwise Operator3/1, Switch/1, Bitwise Operator2/2, Bitwise Operator1/2, Bitwise Operator/2, Product/2, Add2/2, Add4/2, Add1/2, Add/2
  Switch/1 -> Multiport Switch/14  "PASS"
  Multiport Switch/1 -> alu_result/1, MATLAB Function1/3(alu_result), MATLAB Function/3(alu_result), Compare To Zero1/1, Bitwise Operator4/1  "alu_result"
  Constant/1 -> Multiport Switch/34
  alu_a/1 -> MATLAB Function1/1(alu_a), MATLAB Function/1(alu_a), Add4/1, Shift Arithmetic/1, Shift Arithmetic1/1, Subsystem3/1(alu_a), Subsystem6/1(alu_a), Subsystem9/1(alu_a), Subsystem8/1(alu_a), Subsystem7/1(alu_a), Subsystem5/1(alu_a), Subsystem4/1(alu_a), Subsystem2/1(In1), Subsystem1/1(alu_a), Subsystem/1(alu_a), REV16/1(u), Byte Reversal/1, Bitwise Operator8/1, Bit Slice1/1, Bit Slice/1, Data Type Conversion/1, Bitwise Operator6/1, Switch/3, Bitwise Operator5/1, Bitwise Operator2/1, Bitwise Operator1/1, Bitwise Operator/1, Product/1, Add2/1, Add1/1, Add/1
  Product/1 -> Multiport Switch/7  "MUL"
  Bitwise Operator4/1 -> Compare To Zero/1
  Bitwise Operator6/1 -> Multiport Switch/16  "UXTB"
  Constant1/1 -> Bitwise Operator6/2
  Add5/1 -> Multiport Switch/5  "SBC"
  Add2/1 -> Multiport Switch/6  "RSB"
  alu_carry_in/1 -> MATLAB Function/5(alu_carry_in), Logical Operator/1, Add3/2
  Bitwise Operator/1 -> Multiport Switch/8  "AND"
  Add/1 -> Add3/1, Multiport Switch/2  "ADD"
  Logical Operator/1 -> Add5/2
  Bitwise Operator7/1 -> Bitwise Operator5/2
  alu_shamt/1 -> Subsystem9/2("alu_shamt "), Subsystem8/2("alu_shamt "), Shift Arithmetic2/2, Shift Arithmetic1/2, Shift Arithmetic/2
  Bitwise Operator3/1 -> Multiport Switch/12  "MVN"
  Shift Arithmetic1/1 -> Multiport Switch/15  "LSR"
  Bitwise Operator5/1 -> Multiport Switch/11  "BIC"
  Add1/1 -> Multiport Switch/3  "SUB"
  Shift Arithmetic/1 -> Multiport Switch/13  "LSL"
  Bitwise Operator1/1 -> Logical Operator2/1, Multiport Switch/9  "ORR"
  Bitwise Operator2/1 -> Multiport Switch/10  "EOR"
  Constant2/1 -> Bitwise Operator4/2
  Compare To Zero/1 -> alu_n/1  "alu_n"
  Add4/1 -> Add5/1
  Add3/1 -> Multiport Switch/4  "ADC"
  MATLAB Function/1(alu_c) -> alu_c/1  "alu_c"
  alu_src_b/1 -> Switch/2
  Compare To Zero1/1 -> alu_z/1  "alu_z"
  MATLAB Function1/1(alu_v) -> alu_v/1  "alu_v"
  Data Type Conversion/1 -> Shift Arithmetic2/1
  Shift Arithmetic2/1 -> Data Type Conversion1/1
  Data Type Conversion3/1 -> Multiport Switch/18  "SXTH"
  Data Type Conversion6/1 -> Multiport Switch/19  "SXTB"
  Bitwise Operator8/1 -> Multiport Switch/20  "UXTH"
  Data Type Conversion8/1 -> Multiport Switch/21  "REV"
  Subsystem/1(Out1) -> Multiport Switch/23  "REVSH"
  Subsystem1/1(Out1) -> Multiport Switch/24  "MOVT"
  Subsystem3/1(MLS) -> Multiport Switch/26  "MLS"
  Subsystem4/1(MLS) -> Multiport Switch/27  "UMULL"
  Subsystem5/1(MLS) -> Multiport Switch/28  "SMULL"
  Subsystem6/1(MLS) -> Multiport Switch/29  "UDIV"
  Data Type Conversion1/1 -> Multiport Switch/17  "ASR"
  Bit Slice/1 -> Data Type Conversion4/1
  Data Type Conversion4/1 -> Data Type Conversion2/1
  Data Type Conversion2/1 -> Data Type Conversion3/1
  Data Type Conversion7/1 -> Data Type Conversion5/1
  Bit Slice1/1 -> Data Type Conversion7/1
  Data Type Conversion5/1 -> Data Type Conversion6/1
  Constant3/1 -> Bitwise Operator8/2
  Byte Reversal/1 -> Data Type Conversion8/1
  REV16/1(REV16) -> Multiport Switch/22  "REV16"
  Subsystem2/1(MLA) -> Multiport Switch/25  "MLA"
  Subsystem7/1(MLS) -> Multiport Switch/30  "SDIV"
  alu_acc/1 -> Subsystem3/3("alu_acc "), Subsystem2/3("alu_acc ")
  Switch1/1 -> alu_result_hi/1  "alu_result_hi"
  Constant4/1 -> Switch1/3
  Equal/1 -> Logical Operator1/1, Switch2/2  "is_UMULL"
  Equal1/1 -> Logical Operator1/2  "is_SMULL"
  Logical Operator1/1 -> Switch1/2
  Subsystem4/2(MLS1) -> Switch2/1
  Subsystem5/2(MLS1) -> Switch2/3
  [alu_op] -> Equal1/1, Equal/1
  Constant5/1 -> Equal/2
  Constant6/1 -> Equal1/2
  Switch2/1 -> Switch1/1
  Subsystem8/1(MLS1) -> Multiport Switch/31
  Logical Operator2/1 -> Multiport Switch/32  "ORN"
  Subsystem9/1(MLS1) -> Multiport Switch/33  "UBFX"

== system Three_Stages/APSR ==
  alu_c : Inport
  alu_v : Inport  Port=2
  alu_z : Inport  Port=3
  alu_n : Inport  Port=4
  s : Inport  Port=5
  valid : Inport  Port=6
  is_store : Inport  Port=7
  is_load : Inport  Port=8
  Bitwise NOT4 : simulink/Logic and Bit Operations/Bitwise Operator  logicop=NOT  UseBitMask=off  BitMask=bin2dec('11011001')  BitMaskRealWorld=Stored Integer
      settings: LibrarySourceBlock=|
      | simulink/Quick Insert/Logic and Bit
      | Operations/Bitwise NOT
  Bitwise NOT5 : simulink/Logic and Bit Operations/Bitwise Operator  logicop=NOT  UseBitMask=off  BitMask=bin2dec('11011001')  BitMaskRealWorld=Stored Integer
      settings: LibrarySourceBlock=|
      | simulink/Quick Insert/Logic and Bit
      | Operations/Bitwise NOT
  Logical Operator : Logic  Inputs=4  AllPortsSameDT=off  OutDataTypeStr=boolean
  Logical Operator{1..4} (4 alike) : Logic  Operator=NOT  AllPortsSameDT=off  OutDataTypeStr=boolean
  Switch{,1..3} (4 alike) : Switch  Criteria=u2 ~= 0  SaturateOnIntegerOverflow=off  InputSameDT=off
  Unit Delay Enabled Resettable Synchronous{,1..3} (4 alike) : hdlsllib/Discrete/Unit Delay Enabled Resettable Synchronous  InitialCondition=0.0  SampleTime=-1
  apsr_v : Outport
  apsr_z : Outport  Port=2
  apsr_n : Outport  Port=3
  apsr_c : Outport  Port=4
  fwd_c : Outport  Port=5
  fwd_v : Outport  Port=6
  fwd_z : Outport  Port=7
  fwd_n : Outport  Port=8
  wires:
  Bitwise NOT4/1 -> Logical Operator/3
  Logical Operator/1 -> Unit Delay Enabled Resettable Synchronous3/2, Unit Delay Enabled Resettable Synchronous2/2, Unit Delay Enabled Resettable Synchronous1/2, Unit Delay Enabled Resettable Synchronous/2, Switch3/2, Switch2/2, Switch1/2, Switch/2  "fwd_use"
  Unit Delay Enabled Resettable Synchronous1/1 -> apsr_z/1, Switch1/3  "apsr_z"
  valid/1 -> Logical Operator/1
  Unit Delay Enabled Resettable Synchronous2/1 -> apsr_c/1, Switch2/3  "apsr_c"
  alu_z/1 -> Switch1/1, Unit Delay Enabled Resettable Synchronous1/1
  Switch1/1 -> fwd_z/1  "fwd_z"
  Unit Delay Enabled Resettable Synchronous/1 -> apsr_n/1, Switch/3  "apsr_n"
  [rst_n] -> Logical Operator1/1, Logical Operator4/1, Logical Operator3/1, Logical Operator2/1
  Bitwise NOT5/1 -> Logical Operator/4
  alu_v/1 -> Switch3/1, Unit Delay Enabled Resettable Synchronous3/1
  Unit Delay Enabled Resettable Synchronous3/1 -> apsr_v/1, Switch3/3  "apsr_v"
  alu_n/1 -> Switch/1, Unit Delay Enabled Resettable Synchronous/1
  Logical Operator1/1 -> Unit Delay Enabled Resettable Synchronous/3
  alu_c/1 -> Switch2/1, Unit Delay Enabled Resettable Synchronous2/1
  Logical Operator4/1 -> Unit Delay Enabled Resettable Synchronous3/3
  s/1 -> Logical Operator/2
  Logical Operator2/1 -> Unit Delay Enabled Resettable Synchronous1/3
  Logical Operator3/1 -> Unit Delay Enabled Resettable Synchronous2/3
  Switch3/1 -> fwd_v/1  "fwd_v"
  is_load/1 -> Bitwise NOT4/1
  is_store/1 -> Bitwise NOT5/1
  Switch/1 -> fwd_n/1  "fwd_n"
  Switch2/1 -> fwd_c/1  "fwd_c"

== system Three_Stages/Branch_Unit ==
  id_instr3 : Inport  OutDataTypeStr=uint32
  id_instr : Inport  Port=2  OutDataTypeStr=uint32
  id_instr1 : Inport  Port=3  OutDataTypeStr=boolean
  id_instr4 : Inport  Port=4
  id_instr5 : Inport  Port=5
  id_instr6 : Inport  Port=6
  id_instr7 : Inport  Port=7  OutDataTypeStr=uint32
  id_instr8 : Inport  Port=8
  id_instr9 : Inport  Port=9
  id_instr10 : Inport  Port=10
  id_instr11 : Inport  Port=11
  Constant : Constant  Value=0  OutDataTypeStr=uint32
  Constant{1..4} (4 alike) : Constant  OutDataTypeStr=boolean
  Constant5 : Constant  Value=0  OutDataTypeStr=boolean
  Constant6 : Constant  Value=34
  Equal : RelationalOperator  Operator===  OutDataTypeStr=boolean  RndMeth=Simplest  InputSameDT=off
  Logical Operator : Logic  Inputs=3  AllPortsSameDT=off  OutDataTypeStr=boolean
  Multiport Switch : MultiPortSwitch  DataPortOrder=Zero-based contiguous  Inputs=14  DataPortForDefault=Additional data port  DiagnosticForDefault=None  zeroidx=on  SaturateOnIntegerOverflow=off  InputSameDT=off
  Multiport Switch1 : MultiPortSwitch  DataPortOrder=Zero-based contiguous  Inputs=14  DataPortForDefault=Additional data port  DiagnosticForDefault=None  zeroidx=on  SaturateOnIntegerOverflow=off  InputSameDT=off
  Subsystem : Subsystem
      settings: PortSchema="{\"entries\":[{\"content\":{\"sides\":[{\"content\":{\"connectorIds\":[\"In1\",\"In2\",\"In3\",\"In4\",\"In5\",\"In6\",\"In7\",\"In8\",\"In9\",\"In10\",\"In11\"]},\"type\":\"ConnectorPlacement.EquallySpacedRectSide\",\"uuid\":\"55b95d51-a88d-49b0-a57e-406fd3201c21\"},{\"content\":{\"connectorIds\":[\"Out1\",\"Out2\",\"Out3\",\"Out4\",\"Out5\",\"Out6\",\"Out7\"],\"side\":\"RIGHT\"},\"type\":\"ConnectorPlacement.EquallySpacedRectSide\",\"uuid\":\"5df9f469-3634-40eb-b668-079a72bb7c85\"},{\"content\":{\"side\":\"TOP\"},\"type\":\"ConnectorPlacement.EquallySpacedRectSide\",\"uuid\":\"ee959f35-6f67-45be-b7ac-7fdb9e06fb21\"},{\"content\":{\"connectorIds\":[\"Out8\",\"Out9\",\"Out10\"],\"side\":\"BOTTOM\"},\"type\":\"ConnectorPlacement.EquallySpacedRectSide\",\"uuid\":\"61268db3-cc96-4af5-b964-50d53987cff2\"}]},\"type\":\"ConnectorPlacement.EquallySpacedConnector\",\"uuid\":\"636677c6-f4ec-4c64-a5bd-b78980f96ba8\"}],\"packageUris\":[\"http://schema.mathworks.com/mf0/Connector/R2020b\"],\"version\":\"1.0\"}"
  link_en_in : Outport
  Out2 : Outport  Port=2  OutDataTypeStr=uint32
  Out1 : Outport  Port=3  OutDataTypeStr=boolean
  wires:
  Constant/1 -> Multiport Switch/16
  Constant1/1 -> Multiport Switch1/2
  Constant2/1 -> Multiport Switch1/3
  Subsystem/7(target_cbz) -> Multiport Switch/15, Multiport Switch/14
  Subsystem/3(target_bw) -> Multiport Switch/3, Multiport Switch/11
  Subsystem/4(target_bcond) -> Multiport Switch/5, Multiport Switch/4, Multiport Switch/6, Multiport Switch/7, Multiport Switch/8, Multiport Switch/10, Multiport Switch/9
  id_instr/1 -> Subsystem/1(id_instr)  "id_instr"
  id_instr1/1 -> Subsystem/2(id_instr_width)  "id_instr_width"
  Subsystem/2(target_b) -> Multiport Switch/2
  Subsystem/5(target_bl) -> Multiport Switch/12  "target_bl"
  Subsystem/6(target_bx) -> Multiport Switch/13
  Subsystem/10(cond_pass) -> Multiport Switch1/11, Multiport Switch1/10, Multiport Switch1/9, Multiport Switch1/8, Multiport Switch1/7, Multiport Switch1/6, Multiport Switch1/5, Multiport Switch1/4
  Constant3/1 -> Multiport Switch1/12
  Constant4/1 -> Multiport Switch1/13
  Subsystem/9(cbz_taken) -> Multiport Switch1/14
  Subsystem/8(cbnz_taken) -> Multiport Switch1/15
  Constant5/1 -> Multiport Switch1/16
  Multiport Switch1/1 -> Logical Operator/1  "branch_taken"
  Multiport Switch/1 -> Out2/1  "branch_target"
  id_instr5/1 -> Equal/1, Subsystem/5(id_opcode)  "id_opcode"
  Constant6/1 -> Equal/2
  Equal/1 -> link_en_in/1  "id_link_en"
  id_instr3/1 -> Subsystem/3(id_pc)  "id_pc"
  id_instr4/1 -> Logical Operator/2, Subsystem/4(id_valid)  "id_valid"
  id_instr6/1 -> Subsystem/6(id_cond)  "id_cond"
  id_instr7/1 -> Subsystem/7(id_rm_data)  "id_rm_data"
  id_instr8/1 -> Subsystem/8(fwd_z)  "fwd_z"
  id_instr9/1 -> Subsystem/9(fwd_n)  "fwd_n"
  id_instr10/1 -> Subsystem/10(fwd_c)  "fwd_c"
  id_instr11/1 -> Subsystem/11(fwd_v)  "fwd_v"
  Subsystem/1(opcode_sel) -> Multiport Switch/1, Multiport Switch1/1  "opcode_sel"
  [rst_n] -> Logical Operator/3
  Logical Operator/1 -> Out1/1

== system Three_Stages/COND_OK ==
  apsr_v : Inport
  z : Inport  Port=2
  apsr_n : Inport  Port=3
  cf : Inport  Port=4
  cond_out : Inport  Port=5
  Constant : Constant
  Constant1 : Constant
  Logical Operator{,1..3} (4 alike) : Logic  Operator=NOT  AllPortsSameDT=off  OutDataTypeStr=boolean
  Logical Operator4 : Logic  AllPortsSameDT=off  OutDataTypeStr=boolean
  Logical Operator5 : Logic  AllPortsSameDT=off  OutDataTypeStr=boolean
  Logical Operator6 : Logic  Operator=OR  AllPortsSameDT=off  OutDataTypeStr=boolean
  Logical Operator7 : Logic  Operator=OR  AllPortsSameDT=off  OutDataTypeStr=boolean
  Multiport Switch : MultiPortSwitch  DataPortOrder=Zero-based contiguous  Inputs=16  zeroidx=on  SaturateOnIntegerOverflow=off  InputSameDT=off
  Relational Operator : RelationalOperator  Operator=~=  OutDataTypeStr=boolean  RndMeth=Simplest  InputSameDT=off
  Relational Operator1 : RelationalOperator  Operator===  OutDataTypeStr=boolean  RndMeth=Simplest  InputSameDT=off
  Out1 : Outport
  wires:
  z/1 -> Logical Operator7/1, Multiport Switch/2, Logical Operator6/1, Logical Operator/1  "z"
  cf/1 -> Logical Operator1/1, Logical Operator4/2, Multiport Switch/4  "cf"
  apsr_n/1 -> Multiport Switch/6, Logical Operator2/1, Relational Operator1/1, Relational Operator/1  "n"
  apsr_v/1 -> Multiport Switch/8, Relational Operator1/2, Relational Operator/2, Logical Operator3/1  "v"
  Relational Operator/1 -> Multiport Switch/13, Logical Operator7/2  "xor_nv"
  Relational Operator1/1 -> Multiport Switch/12, Logical Operator5/2  "xnor_nv"
  Logical Operator/1 -> Logical Operator4/1, Multiport Switch/3, Logical Operator5/1
  Logical Operator1/1 -> Multiport Switch/5, Logical Operator6/2
  Multiport Switch/1 -> Out1/1  "cond_ok"
  cond_out/1 -> Multiport Switch/1  "ex_cond"
  Logical Operator2/1 -> Multiport Switch/7
  Logical Operator3/1 -> Multiport Switch/9
  Logical Operator4/1 -> Multiport Switch/10
  Logical Operator6/1 -> Multiport Switch/11
  Logical Operator5/1 -> Multiport Switch/14
  Logical Operator7/1 -> Multiport Switch/15
  Constant/1 -> Multiport Switch/16
  Constant1/1 -> Multiport Switch/17

== system Three_Stages/Forward_Unit ==
  note: // Priority: EX same-cycle > EX delayed > MR multi-cycle
  mr_rf_we : Inport
  rf_wdata : Inport  Port=2
  mr_rf_wdata : Inport  Port=3
  mr_rf_addr : Inport  Port=4
  "Forwarding source 1: EX -> ID (same cycle)" : Subsystem
  "Forwarding source 2: MR -> ID (multi-cycle)" : Subsystem
      settings: PortSchema="{\"entries\":[{\"content\":{\"sides\":[{\"content\":{\"connectorIds\":[\"In1\",\"In2\",\"In3\",\"In4\",\"In5\",\"In6\",\"In7\"]},\"type\":\"ConnectorPlacement.EquallySpacedRectSide\",\"uuid\":\"0a06a26d-1e52-4615-b6e3-e87188255e88\"},{\"content\":{\"side\":\"RIGHT\"},\"type\":\"ConnectorPlacement.EquallySpacedRectSide\",\"uuid\":\"5ad7996b-77be-45c8-a933-6eb5d674a378\"},{\"content\":{\"connectorIds\":[\"Out1\",\"Out2\",\"Out3\"],\"side\":\"TOP\"},\"type\":\"ConnectorPlacement.EquallySpacedRectSide\",\"uuid\":\"d808e1bd-bae0-4ea9-b7ce-292750deaaf8\"}]},\"type\":\"ConnectorPlacement.EquallySpacedConnector\",\"uuid\":\"4d2ff6d5-14af-4558-bfdb-0e64c208384f\"}],\"packageUris\":[\"http://schema.mathworks.com/mf0/Connector/R2020b\"],\"version\":\"1.0\"}"
  "Forwarding source 3: EX -> ID (delayed by 1 cycle)" : Subsystem
      settings: PortSchema="{\"entries\":[{\"content\":{\"sides\":[{\"content\":{\"connectorIds\":[\"In1\",\"In2\",\"In3\",\"In4\",\"In5\",\"In6\",\"In7\",\"In8\",\"In9\",\"In10\",\"In11\",\"In12\",\"In13\"]},\"type\":\"ConnectorPlacement.EquallySpacedRectSide\",\"uuid\":\"68bc24ed-b34c-4cba-903a-900180bb9c9b\"},{\"content\":{\"connectorIds\":[\"Out1\",\"Out2\"],\"side\":\"RIGHT\"},\"type\":\"ConnectorPlacement.EquallySpacedRectSide\",\"uuid\":\"d714debd-3431-4e97-8de9-877b62f672f9\"},{\"content\":{\"side\":\"TOP\"},\"type\":\"ConnectorPlacement.EquallySpacedRectSide\",\"uuid\":\"590802f7-6da7-4e93-b71c-e1ba6f396e57\"},{\"content\":{\"connectorIds\":[\"In14\",\"In15\",\"In16\"],\"side\":\"BOTTOM\"},\"type\":\"ConnectorPlacement.EquallySpacedRectSide\",\"uuid\":\"41449ef6-9e5a-4c99-8bb4-61f1257e57e4\"}]},\"type\":\"ConnectorPlacement.EquallySpacedConnector\",\"uuid\":\"dd37a8c8-3bb5-433b-911d-4db9fdfde7c3\"}],\"packageUris\":[\"http://schema.mathworks.com/mf0/Connector/R2020b\"],\"version\":\"1.0\"}"
  id_ex_data_1_in : Outport
  id_ex_data_2_in : Outport  Port=2
  wires:
  "Forwarding source 3: EX -> ID (delayed by 1 cycle)"/2(data_2_in) -> id_ex_data_2_in/1  "id_ex_data_2_in"
  "Forwarding source 1: EX -> ID (same cycle)"/2(Out2) -> "Forwarding source 3: EX -> ID (delayed by 1 cycle)"/2(In8)
  [id_read_addr_2] -> "Forwarding source 2: MR -> ID (multi-cycle)"/7(In28)
  mr_rf_addr/1 -> "Forwarding source 2: MR -> ID (multi-cycle)"/2(rf_addr)
  "Forwarding source 2: MR -> ID (multi-cycle)"/3(Out10) -> "Forwarding source 3: EX -> ID (delayed by 1 cycle)"/16(In14)
  "Forwarding source 2: MR -> ID (multi-cycle)"/2(Out5) -> "Forwarding source 3: EX -> ID (delayed by 1 cycle)"/15(In7)
  [id_read_addr_1] -> "Forwarding source 2: MR -> ID (multi-cycle)"/5(In14)
  [id_read_addr_1] -> "Forwarding source 3: EX -> ID (delayed by 1 cycle)"/9(In4)
  [id_read_en_1] -> "Forwarding source 3: EX -> ID (delayed by 1 cycle)"/8(In3)
  rf_wdata/1 -> "Forwarding source 3: EX -> ID (delayed by 1 cycle)"/3(In2)
  [ex_valid_eff] -> "Forwarding source 3: EX -> ID (delayed by 1 cycle)"/4(In15)
  [id_read_en_2] -> "Forwarding source 2: MR -> ID (multi-cycle)"/6(In27)
  "Forwarding source 1: EX -> ID (same cycle)"/1(Out1) -> "Forwarding source 3: EX -> ID (delayed by 1 cycle)"/1(In1)
  [ex_WB_en_eff] -> "Forwarding source 3: EX -> ID (delayed by 1 cycle)"/5(In16)
  [id_read_addr_2] -> "Forwarding source 3: EX -> ID (delayed by 1 cycle)"/12(In11)
  [ex_is_multi_op] -> "Forwarding source 3: EX -> ID (delayed by 1 cycle)"/6(In17)
  [id_read_data_1] -> "Forwarding source 3: EX -> ID (delayed by 1 cycle)"/10(In5)
  [ex_WB_addr] -> "Forwarding source 3: EX -> ID (delayed by 1 cycle)"/7(In18)
  [id_read_en_2] -> "Forwarding source 3: EX -> ID (delayed by 1 cycle)"/11(In10)
  [id_read_data_2] -> "Forwarding source 3: EX -> ID (delayed by 1 cycle)"/13(In12)
  "Forwarding source 2: MR -> ID (multi-cycle)"/1(Out4) -> "Forwarding source 3: EX -> ID (delayed by 1 cycle)"/14(In6)
  [id_read_en_1] -> "Forwarding source 2: MR -> ID (multi-cycle)"/4(In13)
  mr_rf_we/1 -> "Forwarding source 2: MR -> ID (multi-cycle)"/1(rf_we)
  "Forwarding source 3: EX -> ID (delayed by 1 cycle)"/1(id_instr7) -> id_ex_data_1_in/1  "id_ex_data_1_in"
  mr_rf_wdata/1 -> "Forwarding source 2: MR -> ID (multi-cycle)"/3(rf_wdata)
